simulink model "SR_Stage4"  (R2024b)
settings: Solver=ode4  StartTime=0.0  StopTime=P.Tend  FixedStep=P.Ts  RelTol=1e-3
InitFcn:
  | sr_params; sr_params_stage3; sr_params_stage4; TR = sr_track(P, trackType);
undefined symbols (not defined in the file): P, TR
settings Model: Creator=sange  LastModifiedBy=sange
settings DataIOCC: SaveOutput=off

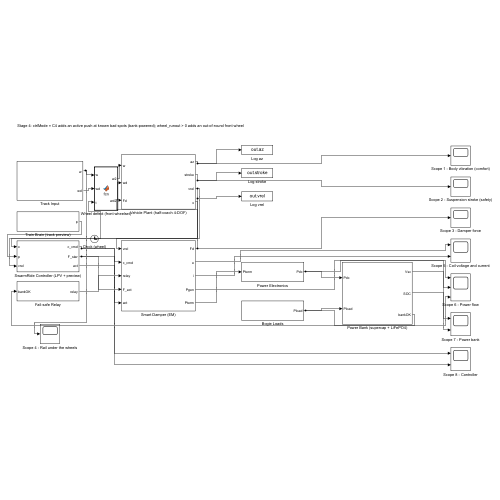
[thumbnail: Simulink's stored preview of the top-level diagram]
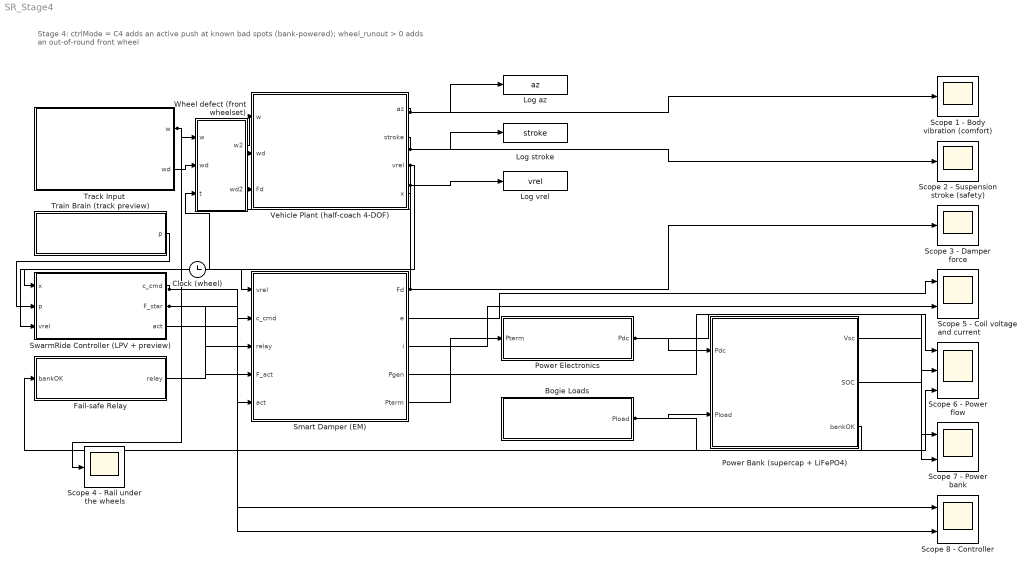
== system SR_Stage4 ==
  note: Stage 4: ctrlMode = C4 adds an active push at known bad spots (bank-powered); wheel_runout > 0 adds an out-of-round front wheel
  Bogie Loads : Subsystem  Description=Electrical loads on each bogie, supplied by the power bank.
  Clock (wheel) : Clock
  Fail-safe Relay : Subsystem  Description=Drops the relay (coil connected to the fail-safe resistor) on a fault or when the power bank cannot run the controller. The damper then behaves like today's passive damper.
  Log az : ToWorkspace  VariableName=az  SaveFormat=Timeseries  SampleTime=P.Ts
  Log stroke : ToWorkspace  VariableName=stroke  SaveFormat=Timeseries  SampleTime=P.Ts
  Log vrel : ToWorkspace  VariableName=vrel  SaveFormat=Timeseries  SampleTime=P.Ts
  Power Bank (supercap + LiFePO4) : Subsystem  Description=Supercapacitor catches the short power bursts; the LiFePO4 battery stores energy; the energy supervisor decides where the power goes (instead of a Stateflow chart).
  Power Electronics : Subsystem  Description=Average models of the power stages. The rectifier turns the coil's AC into DC; the DC-DC converter raises the voltage to charge the bank. Each loses a few percent; neither adds energy.
  Scope 1 - Body vibration (comfort) : Scope
  Scope 2 - Suspension stroke (safety) : Scope
  Scope 3 - Damper force : Scope
  Scope 4 - Rail under the wheels : Scope
  Scope 5 - Coil voltage and current : Scope  NumInputPorts=2
  Scope 6 - Power flow : Scope  NumInputPorts=3
  Scope 7 - Power bank : Scope  NumInputPorts=2
  Scope 8 - Controller : Scope  NumInputPorts=2
  Smart Damper (EM) : Subsystem  Description=Electromagnetic damper per bogie: e = Ke v, F = Ke i. The H-bridge sets the coil current, and the current sets the damping. Plus the passive part (oil, friction, inertance).
  SwarmRide Controller (LPV + preview) : Subsystem  Description=LPV state feedback (gains blended by measured load) plus Train Brain preview feed-forward, converted to a damping command the damper can give (resist only, efficiency limit).
  Track Input : Subsystem  Description=Generates the vertical rail irregularity under each of the 4 wheels. Each wheel sees the same rail, delayed by its distance behind the lead wheel.
  Train Brain (track preview) : Subsystem  Description=Rail profile around the lead wheel, from the fleet track map and the locomotive's lead bogie: one sample every Tc of travel, 1 s ahead. preview_dt shifts it in time.
  Vehicle Plant (half-coach 4-DOF) : Subsystem  Description=Coach body (bounce + pitch) on two bogies. Secondary suspension = air spring (inside the equations) + damper force Fd (input). Primary suspension = springs + dampers to 4 wheelsets.
  Wheel defect (front wheelset) : MATLAB Function  TreatAsAtomicUnit=on
  wires:
  Track Input/1(w) -> Scope 4 - Rail under the wheels/1, Wheel defect (front wheelset)/1(w)
  Vehicle Plant (half-coach 4-DOF)/3(vrel) -> Smart Damper (EM)/1(vrel), Log vrel/1, SwarmRide Controller (LPV + preview)/3(vrel)
  Fail-safe Relay/1(relay) -> Smart Damper (EM)/3(relay)
  Smart Damper (EM)/1(Fd) -> Vehicle Plant (half-coach 4-DOF)/3(Fd), Scope 3 - Damper force/1
  Smart Damper (EM)/5(Pterm) -> Power Electronics/1(Pterm)
  Power Electronics/1(Pdc) -> Power Bank (supercap + LiFePO4)/1(Pdc), Scope 6 - Power flow/2
  Bogie Loads/1(Pload) -> Power Bank (supercap + LiFePO4)/2(Pload), Scope 6 - Power flow/3
  Power Bank (supercap + LiFePO4)/3(bankOK) -> Fail-safe Relay/1(bankOK)
  Vehicle Plant (half-coach 4-DOF)/1(az) -> Log az/1, Scope 1 - Body vibration (comfort)/1
  Vehicle Plant (half-coach 4-DOF)/2(stroke) -> Log stroke/1, Scope 2 - Suspension stroke (safety)/1
  Smart Damper (EM)/2(e) -> Scope 5 - Coil voltage and current/1
  Smart Damper (EM)/3(i) -> Scope 5 - Coil voltage and current/2
  Smart Damper (EM)/4(Pgen) -> Scope 6 - Power flow/1
  Power Bank (supercap + LiFePO4)/1(Vsc) -> Scope 7 - Power bank/1
  Power Bank (supercap + LiFePO4)/2(SOC) -> Scope 7 - Power bank/2
  Vehicle Plant (half-coach 4-DOF)/4(x) -> SwarmRide Controller (LPV + preview)/1(x)
  Train Brain (track preview)/1(p) -> SwarmRide Controller (LPV + preview)/2(p)
  SwarmRide Controller (LPV + preview)/1(c_cmd) -> Smart Damper (EM)/2(c_cmd), Scope 8 - Controller/2
  SwarmRide Controller (LPV + preview)/2(F_star) -> Scope 8 - Controller/1, Smart Damper (EM)/4(F_act)
  SwarmRide Controller (LPV + preview)/3(act) -> Smart Damper (EM)/5(act)
  Track Input/2(wd) -> Wheel defect (front wheelset)/2(wd)
  Clock (wheel)/1 -> Wheel defect (front wheelset)/3(t)
  Wheel defect (front wheelset)/1(w2) -> Vehicle Plant (half-coach 4-DOF)/1(w)
  Wheel defect (front wheelset)/2(wd2) -> Vehicle Plant (half-coach 4-DOF)/2(wd)

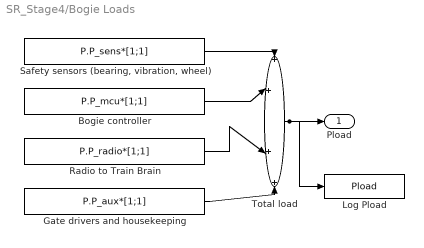
== system SR_Stage4/Bogie Loads ==
  Bogie controller : Constant  Value=P.P_mcu*[1;1]  SampleTime=P.Ts
  Gate drivers and housekeeping : Constant  Value=P.P_aux*[1;1]  SampleTime=P.Ts
  Log Pload : ToWorkspace  VariableName=Pload  SaveFormat=Timeseries  SampleTime=P.Ts
  Radio to Train Brain : Constant  Value=P.P_radio*[1;1]  SampleTime=P.Ts
  "Safety sensors (bearing, vibration, wheel)" : Constant  Value=P.P_sens*[1;1]  SampleTime=P.Ts
  Total load : Sum  Inputs=++++
  Pload : Outport
  wires:
  "Safety sensors (bearing, vibration, wheel)"/1 -> Total load/1
  Bogie controller/1 -> Total load/2
  Radio to Train Brain/1 -> Total load/3
  Gate drivers and housekeeping/1 -> Total load/4
  Total load/1 -> Pload/1, Log Pload/1

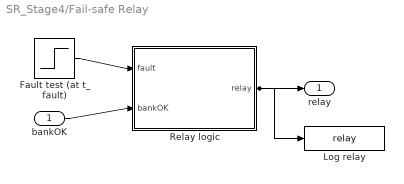
== system SR_Stage4/Fail-safe Relay ==
  bankOK : Inport
  Fault test (at t_fault) : Step  Time=P.t_fault  SampleTime=0
  Log relay : ToWorkspace  VariableName=relay  SaveFormat=Timeseries  SampleTime=P.Ts
  Relay logic : MATLAB Function  TreatAsAtomicUnit=on
  relay : Outport
  wires:
  Fault test (at t_fault)/1 -> Relay logic/1(fault)
  bankOK/1 -> Relay logic/2(bankOK)
  Relay logic/1(relay) -> relay/1, Log relay/1

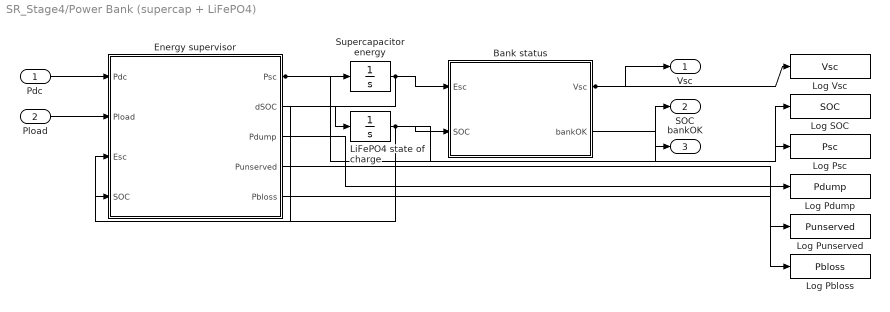
== system SR_Stage4/Power Bank (supercap + LiFePO4) ==
  Pdc : Inport
  Pload : Inport  Port=2
  Bank status : MATLAB Function  TreatAsAtomicUnit=on
  Energy supervisor : MATLAB Function  TreatAsAtomicUnit=on
  LiFePO4 state of charge : Integrator  InitialCondition=P.SOC0*[1;1]
  Log Pbloss : ToWorkspace  VariableName=Pbloss  SaveFormat=Timeseries  SampleTime=P.Ts
  Log Pdump : ToWorkspace  VariableName=Pdump  SaveFormat=Timeseries  SampleTime=P.Ts
  Log Psc : ToWorkspace  VariableName=Psc  SaveFormat=Timeseries  SampleTime=P.Ts
  Log Punserved : ToWorkspace  VariableName=Punserved  SaveFormat=Timeseries  SampleTime=P.Ts
  Log SOC : ToWorkspace  VariableName=SOC  SaveFormat=Timeseries  SampleTime=P.Ts
  Log Vsc : ToWorkspace  VariableName=Vsc  SaveFormat=Timeseries  SampleTime=P.Ts
  Supercapacitor energy : Integrator  InitialCondition=P.Esc0*[1;1]
  Vsc : Outport
  SOC : Outport  Port=2
  bankOK : Outport  Port=3
  wires:
  Pdc/1 -> Energy supervisor/1(Pdc)
  Pload/1 -> Energy supervisor/2(Pload)
  Supercapacitor energy/1 -> Energy supervisor/3(Esc), Bank status/1(Esc)
  LiFePO4 state of charge/1 -> Energy supervisor/4(SOC), Bank status/2(SOC), SOC/1, Log SOC/1
  Energy supervisor/1(Psc) -> Supercapacitor energy/1, Log Psc/1
  Energy supervisor/2(dSOC) -> LiFePO4 state of charge/1
  Bank status/1(Vsc) -> Vsc/1, Log Vsc/1
  Bank status/2(bankOK) -> bankOK/1
  Energy supervisor/3(Pdump) -> Log Pdump/1
  Energy supervisor/4(Punserved) -> Log Punserved/1
  Energy supervisor/5(Pbloss) -> Log Pbloss/1

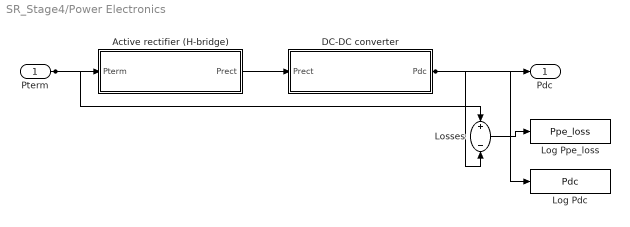
== system SR_Stage4/Power Electronics ==
  Pterm : Inport
  Active rectifier (H-bridge) : MATLAB Function  TreatAsAtomicUnit=on
  DC-DC converter : MATLAB Function  TreatAsAtomicUnit=on
  Log Pdc : ToWorkspace  VariableName=Pdc  SaveFormat=Timeseries  SampleTime=P.Ts
  Log Ppe_loss : ToWorkspace  VariableName=Ppe_loss  SaveFormat=Timeseries  SampleTime=P.Ts
  Losses : Sum  Inputs=+-
  Pdc : Outport
  wires:
  Pterm/1 -> Active rectifier (H-bridge)/1(Pterm), Losses/1
  Active rectifier (H-bridge)/1(Prect) -> DC-DC converter/1(Prect)
  DC-DC converter/1(Pdc) -> Pdc/1, Losses/2, Log Pdc/1
  Losses/1 -> Log Ppe_loss/1

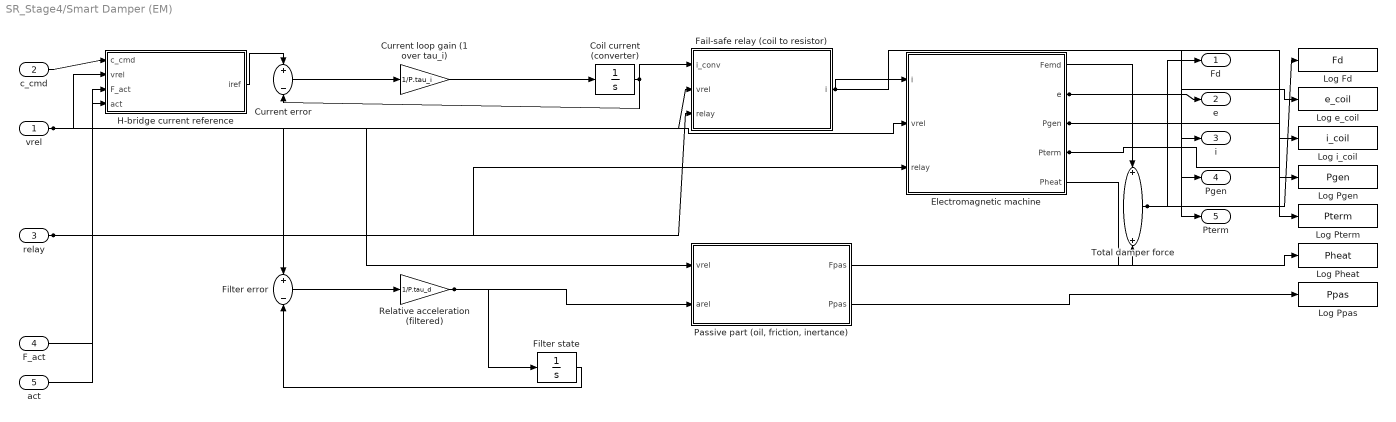
== system SR_Stage4/Smart Damper (EM) ==
  vrel : Inport
  c_cmd : Inport  Port=2
  relay : Inport  Port=3
  F_act : Inport  Port=4
  act : Inport  Port=5
  Coil current (converter) : Integrator  InitialCondition=zeros(2,1)
  Current error : Sum  Inputs=+-
  Current loop gain (1 over tau_i) : Gain  Gain=1/P.tau_i
  Electromagnetic machine : MATLAB Function  TreatAsAtomicUnit=on
  Fail-safe relay (coil to resistor) : MATLAB Function  TreatAsAtomicUnit=on
  Filter error : Sum  Inputs=+-
  Filter state : Integrator  InitialCondition=zeros(2,1)
  H-bridge current reference : MATLAB Function  TreatAsAtomicUnit=on
  Log Fd : ToWorkspace  VariableName=Fd  SaveFormat=Timeseries  SampleTime=P.Ts
  Log Pgen : ToWorkspace  VariableName=Pgen  SaveFormat=Timeseries  SampleTime=P.Ts
  Log Pheat : ToWorkspace  VariableName=Pheat  SaveFormat=Timeseries  SampleTime=P.Ts
  Log Ppas : ToWorkspace  VariableName=Ppas  SaveFormat=Timeseries  SampleTime=P.Ts
  Log Pterm : ToWorkspace  VariableName=Pterm  SaveFormat=Timeseries  SampleTime=P.Ts
  Log e_coil : ToWorkspace  VariableName=e_coil  SaveFormat=Timeseries  SampleTime=P.Ts
  Log i_coil : ToWorkspace  VariableName=i_coil  SaveFormat=Timeseries  SampleTime=P.Ts
  "Passive part (oil, friction, inertance)" : MATLAB Function  TreatAsAtomicUnit=on
  Relative acceleration (filtered) : Gain  Gain=1/P.tau_d
  Total damper force : Sum
  Fd : Outport
  e : Outport  Port=2
  i : Outport  Port=3
  Pgen : Outport  Port=4
  Pterm : Outport  Port=5
  wires:
  c_cmd/1 -> H-bridge current reference/1(c_cmd)
  vrel/1 -> H-bridge current reference/2(vrel), Fail-safe relay (coil to resistor)/2(vrel), Electromagnetic machine/2(vrel), Filter error/1, "Passive part (oil, friction, inertance)"/1(vrel)
  H-bridge current reference/1(iref) -> Current error/1
  Current error/1 -> Current loop gain (1 over tau_i)/1
  Current loop gain (1 over tau_i)/1 -> Coil current (converter)/1
  Coil current (converter)/1 -> Current error/2, Fail-safe relay (coil to resistor)/1(i_conv)
  relay/1 -> Fail-safe relay (coil to resistor)/3(relay), Electromagnetic machine/3(relay)
  Fail-safe relay (coil to resistor)/1(i) -> Electromagnetic machine/1(i), i/1, Log i_coil/1
  Filter error/1 -> Relative acceleration (filtered)/1
  Relative acceleration (filtered)/1 -> Filter state/1, "Passive part (oil, friction, inertance)"/2(arel)
  Filter state/1 -> Filter error/2
  Electromagnetic machine/1(Femd) -> Total damper force/1
  "Passive part (oil, friction, inertance)"/1(Fpas) -> Total damper force/2
  Total damper force/1 -> Fd/1, Log Fd/1
  Electromagnetic machine/2(e) -> e/1, Log e_coil/1
  Electromagnetic machine/3(Pgen) -> Pgen/1, Log Pgen/1
  Electromagnetic machine/4(Pterm) -> Pterm/1, Log Pterm/1
  Electromagnetic machine/5(Pheat) -> Log Pheat/1
  "Passive part (oil, friction, inertance)"/2(Ppas) -> Log Ppas/1
  F_act/1 -> H-bridge current reference/3(F_act)
  act/1 -> H-bridge current reference/4(act)

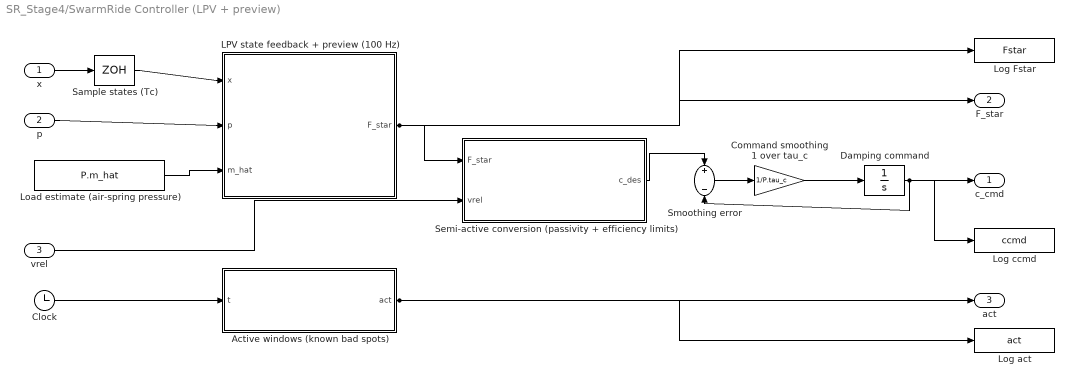
== system SR_Stage4/SwarmRide Controller (LPV + preview) ==
  x : Inport
  p : Inport  Port=2
  vrel : Inport  Port=3
  Active windows (known bad spots) : MATLAB Function  TreatAsAtomicUnit=on
  Clock : Clock
  Command smoothing 1 over tau_c : Gain  Gain=1/P.tau_c
  Damping command : Integrator  InitialCondition=zeros(2,1)
  LPV state feedback + preview (100 Hz) : MATLAB Function  TreatAsAtomicUnit=on
  Load estimate (air-spring pressure) : Constant  Value=P.m_hat  SampleTime=P.Tc
  Log Fstar : ToWorkspace  VariableName=Fstar  SaveFormat=Timeseries  SampleTime=P.Ts
  Log act : ToWorkspace  VariableName=act  SaveFormat=Timeseries  SampleTime=P.Ts
  Log ccmd : ToWorkspace  VariableName=ccmd  SaveFormat=Timeseries  SampleTime=P.Ts
  Sample states (Tc) : ZeroOrderHold  SampleTime=P.Tc
  Semi-active conversion (passivity + efficiency limits) : MATLAB Function  TreatAsAtomicUnit=on
  Smoothing error : Sum  Inputs=+-
  c_cmd : Outport
  F_star : Outport  Port=2
  act : Outport  Port=3
  wires:
  x/1 -> Sample states (Tc)/1
  Sample states (Tc)/1 -> LPV state feedback + preview (100 Hz)/1(x)
  p/1 -> LPV state feedback + preview (100 Hz)/2(p)
  Load estimate (air-spring pressure)/1 -> LPV state feedback + preview (100 Hz)/3(m_hat)
  LPV state feedback + preview (100 Hz)/1(F_star) -> Semi-active conversion (passivity + efficiency limits)/1(F_star), F_star/1, Log Fstar/1
  vrel/1 -> Semi-active conversion (passivity + efficiency limits)/2(vrel)
  Semi-active conversion (passivity + efficiency limits)/1(c_des) -> Smoothing error/1
  Smoothing error/1 -> Command smoothing 1 over tau_c/1
  Command smoothing 1 over tau_c/1 -> Damping command/1
  Damping command/1 -> Smoothing error/2, c_cmd/1, Log ccmd/1
  Clock/1 -> Active windows (known bad spots)/1(t)
  Active windows (known bad spots)/1(act) -> act/1, Log act/1

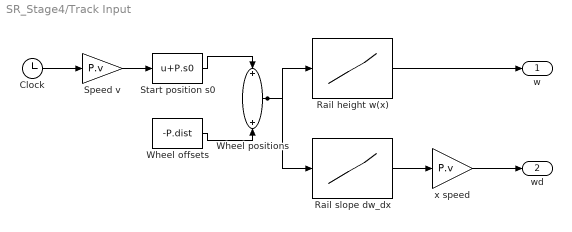
== system SR_Stage4/Track Input ==
  Clock : Clock
  Rail height w(x) : Lookup_n-D  NumberOfTableDimensions=1  BreakpointsForDimension1=TR.x  Table=TR.w  ExtrapMethod=Clip  InternalRulePriority=Speed  RndMeth=Simplest
  Rail slope dw_dx : Lookup_n-D  NumberOfTableDimensions=1  BreakpointsForDimension1=TR.x  Table=TR.dwdx  ExtrapMethod=Clip  InternalRulePriority=Speed  RndMeth=Simplest
  Speed v : Gain  Gain=P.v
  Start position s0 : Bias  Bias=P.s0  SaturateOnIntegerOverflow=off
  Wheel offsets : Constant  Value=-P.dist
  Wheel positions : Sum
  x speed : Gain  Gain=P.v
  w : Outport
  wd : Outport  Port=2
  wires:
  Clock/1 -> Speed v/1
  Speed v/1 -> Start position s0/1
  Start position s0/1 -> Wheel positions/1
  Wheel offsets/1 -> Wheel positions/2
  Wheel positions/1 -> Rail height w(x)/1, Rail slope dw_dx/1
  Rail height w(x)/1 -> w/1
  Rail slope dw_dx/1 -> x speed/1
  x speed/1 -> wd/1

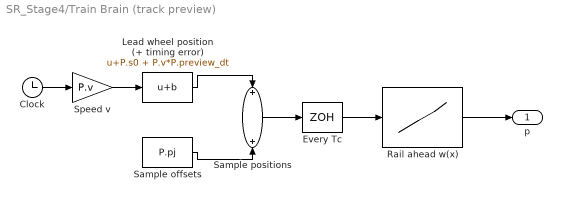
== system SR_Stage4/Train Brain (track preview) ==
  Clock : Clock
  Every Tc : ZeroOrderHold  SampleTime=P.Tc
  Lead wheel position (+ timing error) : Bias  Bias=P.s0 + P.v*P.preview_dt  SaturateOnIntegerOverflow=off
  Rail ahead w(x) : Lookup_n-D  NumberOfTableDimensions=1  BreakpointsForDimension1=TR.x  Table=TR.w  ExtrapMethod=Clip  InternalRulePriority=Speed  RndMeth=Simplest
  Sample offsets : Constant  Value=P.pj
  Sample positions : Sum
  Speed v : Gain  Gain=P.v
  p : Outport
  wires:
  Clock/1 -> Speed v/1
  Speed v/1 -> Lead wheel position (+ timing error)/1
  Lead wheel position (+ timing error)/1 -> Sample positions/1
  Sample offsets/1 -> Sample positions/2
  Sample positions/1 -> Every Tc/1
  Every Tc/1 -> Rail ahead w(x)/1
  Rail ahead w(x)/1 -> p/1

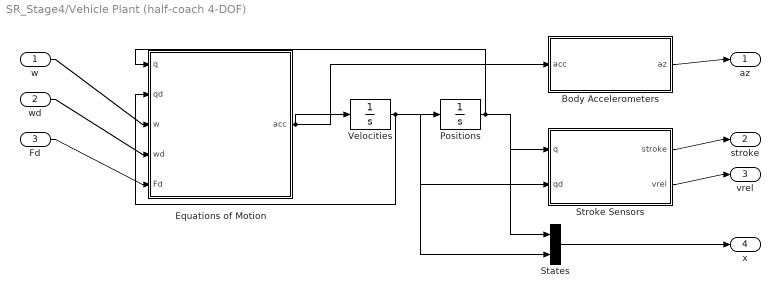
== system SR_Stage4/Vehicle Plant (half-coach 4-DOF) ==
  w : Inport
  wd : Inport  Port=2
  Fd : Inport  Port=3
  Body Accelerometers : MATLAB Function  TreatAsAtomicUnit=on
  Equations of Motion : MATLAB Function  TreatAsAtomicUnit=on
  Positions : Integrator  InitialCondition=zeros(4,1)
  States : Concatenate
  Stroke Sensors : MATLAB Function  TreatAsAtomicUnit=on
  Velocities : Integrator  InitialCondition=zeros(4,1)
  az : Outport
  stroke : Outport  Port=2
  vrel : Outport  Port=3
  x : Outport  Port=4
  wires:
  Positions/1 -> Equations of Motion/1(q), Stroke Sensors/1(q), States/1
  Velocities/1 -> Equations of Motion/2(qd), Positions/1, Stroke Sensors/2(qd), States/2
  w/1 -> Equations of Motion/3(w)
  wd/1 -> Equations of Motion/4(wd)
  Fd/1 -> Equations of Motion/5(Fd)
  Equations of Motion/1(acc) -> Velocities/1, Body Accelerometers/1(acc)
  Body Accelerometers/1(az) -> az/1
  Stroke Sensors/1(stroke) -> stroke/1
  Stroke Sensors/2(vrel) -> vrel/1
  States/1 -> x/1

== matlab function SR_Stage4/Power Electronics/DC-DC converter ==
  data: Prect input; Pdc output size=[2 1]; P parameter
function Pdc = fcn(Prect, P)
% Raises the voltage to the bank voltage. Power out = efficiency x power in (voltage up, current down).
Pdc = P.eta_dcdc * max(Prect, 0) + min(Prect, 0) / P.eta_dcdc;

== matlab function SR_Stage4/Power Bank (supercap + LiFePO4)/Energy supervisor ==
  data: Pdc input; Psc output size=[2 1]; Pload input; Esc input; SOC input; dSOC output size=[2 1]; Pdump output size=[2 1]; Punserved output size=[2 1]; Pbloss output size=[2 1]; P parameter
function [Psc, dSOC, Pdump, Punserved, Pbloss] = fcn(Pdc, Pload, Esc, SOC, P)
% Rules, per bogie:
%  1. Loads and harvested power meet on the supercapacitor (DC link).
%  2. Supercap high (> Vchg): charge the battery.  Supercap low (< Vdis): battery supports.
%  3. Supercap full and battery full: dump the surplus (resistor).
%  4. Supercap empty and battery empty: loads cannot be served.
Psc = zeros(2,1); dSOC = zeros(2,1); Pdump = zeros(2,1); Punserved = zeros(2,1); Pbloss = zeros(2,1);
for b = 1:2
    V = sqrt(max(2 * Esc(b) / P.Csc, 0));
    Pch = 0; Pdis = 0;
    if V > P.Vchg && SOC(b) < P.SOCmax
        Pch = min(P.Pch_max, P.Kv * (V - P.Vchg));
    elseif V < P.Vdis && SOC(b) > P.SOCmin
        Pdis = min(P.Pdis_max, P.Kv * (P.Vdis - V));
    end
    p = Pdc(b) - Pload(b) - Pch + Pdis;
    if V >= P.Vmax && p > 0, Pdump(b) = p; p = 0; end
    if V <= P.Vmin && p < 0, Punserved(b) = -p; p = 0; end
    Psc(b) = p;
    dSOC(b) = (P.eta_ch * Pch - Pdis / P.eta_dis) / (P.Ebat_Wh * 3600);
    Pbloss(b) = (1 - P.eta_ch) * Pch + (1 / P.eta_dis - 1) * Pdis;
end

== matlab function SR_Stage4/Power Bank (supercap + LiFePO4)/Bank status ==
  data: Esc input; Vsc output size=[2 1]; SOC input; bankOK output size=[2 1]; P parameter
function [Vsc, bankOK] = fcn(Esc, SOC, P)
% Supercap voltage from its energy (E = C V^2 / 2); bank OK while either store can run the loads.
Vsc = sqrt(max(2 * Esc / P.Csc, 0));
bankOK = double((Vsc > P.Vmin) | (SOC > P.SOCmin));

== matlab function SR_Stage4/SwarmRide Controller (LPV + preview)/LPV state feedback + preview (100 Hz) ==
  data: x input; F_star output size=[2 1]; p input size=[221 1]; m_hat input; P parameter
function F_star = fcn(x, p, m_hat, P)
% LPV: blend the gains of the two load-grid points around the measured load.
% C2: F* = -Kx x.   C3 / C4: F* = -Kx x - Kp p  (Train Brain preview of the rail around the train).
mg = P.Kgrid_m;  nL = numel(mg);
i = 1;  a = 0;
if m_hat >= mg(nL)
    i = nL - 1;  a = 1;
elseif m_hat > mg(1)
    for k = 1:nL - 1
        if m_hat >= mg(k) && m_hat <= mg(k + 1)
            i = k;  a = (m_hat - mg(k)) / (mg(k + 1) - mg(k));
        end
    end
end
Kx = reshape((1 - a) * P.Kx(i, :) + a * P.Kx(i + 1, :), 2, 8);
F_star = -Kx * x;
if P.ctrl >= 3
    np = size(P.Kp, 2) / 2;
    Kp = reshape((1 - a) * P.Kp(i, :) + a * P.Kp(i + 1, :), 2, np);
    F_star = F_star - Kp * p;
end

== matlab function SR_Stage4/SwarmRide Controller (LPV + preview)/Semi-active conversion (passivity + efficiency limits) ==
  data: F_star input; c_des output size=[2 1]; vrel input; P parameter
function c_des = fcn(F_star, vrel, P)
% The damper can only resist motion, so c = F*/v must be >= 0. It is kept at or below c_cap
% so the coil stays efficient (efficiency >= 1 - c_cap/c_max), and at or above an optional
% floor c_floor that trades comfort for power. C1 uses one fixed setting.
if P.ctrl == 1
    c_des = P.c_fix * ones(2, 1);
else
    c_des = F_star .* vrel ./ (vrel.^2 + P.eps_v^2) - P.c_oil;
    c_des = min(max(c_des, P.c_floor), P.c_cap);
end

== matlab function SR_Stage4/Vehicle Plant (half-coach 4-DOF)/Body Accelerometers ==
  data: acc input; az output size=[3 1]; P parameter
function az = fcn(acc, P)
% Body acceleration at the centre and above each bogie (comfort).
az = sr_measure(zeros(4,1), zeros(4,1), acc, P);

== matlab function SR_Stage4/SwarmRide Controller (LPV + preview)/Active windows (known bad spots) ==
  data: t input; act output size=[2 1]; P parameter
function act = fcn(t, P)
% C4 only: 1 while a bogie centre is within the window around a known bad spot from the
% fleet track map; there the damper may push, using energy from the bogie bank.
act = zeros(2, 1);
if P.ctrl == 4
    s  = P.s0 + P.v * t;                          % lead wheel position [m]
    sb = s - [P.ab; 2 * P.lb + P.ab];             % front and rear bogie centres [m]
    for b = 1:2
        for k = 1:numel(P.bad_x)
            if sb(b) >= P.bad_x(k) - P.act_before && sb(b) <= P.bad_x(k) + P.bad_len(k) + P.act_after
                act(b) = 1;
            end
        end
    end
end

== matlab function SR_Stage4/Wheel defect (front wheelset) ==
  data: w input; w2 output size=[4 1]; wd input; t input; wd2 output size=[4 1]; P parameter
function [w2, wd2] = fcn(w, wd, t, P)
% Out-of-round front wheelset: radial run-out of order n raises and lowers the wheel centre
% n times per revolution. Off when P.wheel_runout = 0.
w2 = w;  wd2 = wd;
if P.wheel_runout > 0
    s  = P.s0 + P.v * t;                          % rolling distance of the lead wheel [m]
    ph = P.wheel_order * s / P.wheel_R;
    w2(1)  = w(1) + P.wheel_runout * sin(ph);
    wd2(1) = wd(1) + P.wheel_runout * P.wheel_order * P.v / P.wheel_R * cos(ph);
end

== matlab function SR_Stage4/Vehicle Plant (half-coach 4-DOF)/Equations of Motion ==
  data: q input; acc output size=[4 1]; qd input; w input; wd input; Fd input; P parameter
function acc = fcn(q, qd, w, wd, Fd, P)
% Newton's law for body bounce, body pitch and the two bogie frames.
acc = sr_eom(q, qd, w, wd, Fd, P);

== matlab function SR_Stage4/Vehicle Plant (half-coach 4-DOF)/Stroke Sensors ==
  data: q input; stroke output size=[2 1]; qd input; vrel output size=[2 1]; P parameter
function [stroke, vrel] = fcn(q, qd, P)
% Suspension stroke (safety) and stroke velocity (what the damper feels).
[~, stroke, vrel] = sr_measure(q, qd, zeros(4,1), P);

== matlab function SR_Stage4/Fail-safe Relay/Relay logic ==
  data: fault input; relay output size=[2 1]; bankOK input
function relay = fcn(fault, bankOK)
% 1 = relay dropped: coil on the fail-safe resistor (passive damper). 0 = normal (converter).
relay = double((fault > 0.5) | (bankOK < 0.5));

== matlab function SR_Stage4/Smart Damper (EM)/H-bridge current reference ==
  data: c_cmd input; iref output size=[2 1]; vrel input; F_act input; act input; P parameter
function iref = fcn(c_cmd, vrel, F_act, act, P)
% Normal (semi-active): the current sets the damping, F = nd Ke i = c vrel, c in 0..Ke^2/Rc.
% Inside a C4 window (act = 1): follow the ideal force F* directly. The H-bridge then runs the
% coil as a motor when F* pushes, drawing power from the bank. Current is limited to the rating.
c = min(max(c_cmd, 0), P.cmax_emd);
iref = c .* vrel / (P.nd * P.Ke);
iref = (1 - act) .* iref + act .* F_act / (P.nd * P.Ke);
iref = min(max(iref, -P.imax), P.imax);

== matlab function SR_Stage4/Smart Damper (EM)/Fail-safe relay (coil to resistor) ==
  data: i_conv input; i output size=[2 1]; vrel input; relay input; P parameter
function i = fcn(i_conv, vrel, relay, P)
% Normal: the converter sets the current. Relay dropped: the coil drives the fail-safe resistor.
i_fs = P.Ke * vrel / (P.Rc + P.R_fs);
i = (1 - relay) .* i_conv + relay .* i_fs;

== matlab function SR_Stage4/Smart Damper (EM)/Electromagnetic machine ==
  data: i input; Femd output size=[2 1]; vrel input; relay input; e output size=[2 1]; Pgen output size=[2 1]; Pterm output size=[2 1]; Pheat output size=[2 1]; P parameter
function [Femd, e, Pgen, Pterm, Pheat] = fcn(i, vrel, relay, P)
% Faraday: e = Ke v.  Lorentz: F = Ke i.  nd dampers per bogie.
e     = P.Ke * vrel;                       % back-EMF of one damper [V]
Femd  = P.nd * P.Ke * i;                   % force per bogie [N]
Pgen  = Femd .* vrel;                      % mechanical power converted [W]
Pcu   = P.nd * P.Rc * i.^2;                % coil copper loss [W]
Pfs   = relay .* (P.nd * P.R_fs * i.^2);   % fail-safe resistor heat [W]
Pterm = (1 - relay) .* (Pgen - Pcu);       % electrical power to the converter [W]
Pheat = Pcu + Pfs;

== matlab function SR_Stage4/Smart Damper (EM)/Passive part (oil, friction, inertance) ==
  data: vrel input; Fpas output size=[2 1]; arel input; Ppas output size=[2 1]; P parameter
function [Fpas, Ppas] = fcn(vrel, arel, P)
% Design B: half-size oil damper or Casnub wedges. Design C: screw friction + rotor inertance.
Fdis = P.c_oil * vrel + (P.Ffr2 + P.nd * P.Fc) * tanh(vrel / P.veps);
Fpas = Fdis + P.nd * P.b_in * arel;
Ppas = Fdis .* vrel;                       % heat in the passive part [W]

== matlab function SR_Stage4/Power Electronics/Active rectifier (H-bridge) ==
  data: Pterm input; Prect output size=[2 1]; P parameter
function Prect = fcn(Pterm, P)
% Power out of the rectifier; when power flows backwards (current lag) the losses are on the other side.
Prect = P.eta_rect * max(Pterm, 0) + min(Pterm, 0) / P.eta_rect;
